simulink model "turbo_controller"  (R2025a)
settings: Solver=FixedStepAuto  StartTime=0.0  StopTime=inf  FixedStep=0.001  RelTol=1e-3
PostLoadFcn:
  | % 自动定位同目录CubeMX文件；不需要外部初始化脚本。
  | codertarget.data.setParameterValue('turbo_controller','STM32CubeMX.ProjectFile',fullfile(fileparts(get_param('turbo_controller','FileName')),'turbo_f407.ioc'));
InitFcn:
  | % 中文说明：按原控制器字段与类型创建三组接口总线；控制参数已内嵌。
  | tc_names=["EValve_Cycle" "EValve_Open" "Eblast_Cycle" "Eblast_Open" "Motor_Cycle" "Motor_Open" "EValve_Enable" "Eblast_Enable" "Motor_Enable" "SWO_Firework" "SWO_BleedAir" "EngineState" "Flag_ECUReset_Clear" "Flag_ECUReset_Save" "Flag_Reset_Enable" "Accelerator" "Nc_dem" "Nc"]; tc_types=["uint16" "uint16" "uint16" "uint16" "uint16" "uint16" "uint8" "uint8" "uint8" "uint8" "uint8" "uint8" "uint8" "uint8" "uint8" "single" "single" "single"];
  | for tc_k=1:numel(tc_names)
  |  tc_e(tc_k)=Simulink.BusElement; tc_e(tc_k).Name=char(tc_names(tc_k)); tc_e(tc_k).DataType=char(tc_types(tc_k));
  | end
  | EngineControl_Out=Simulink.Bus; EngineControl_Out.DataScope='Exported'; EngineControl_Out.Elements=tc_e;
  | clear tc_e tc_names tc_types tc_k
  | tc_names=["savedata1" "savedata2" "savedata3" "savedata4" "savedata5" "savedata6" "savedata7" "savedata8" "savedata9" "savedata10" "savedata11" "savedata12" "savedata13" "savedata14" "savedata15" "savedata16" "savedata17" "savedata18" "savedata19" "savedata20" "savedata21" "savedata22" "savedata23" "savedata24" "savedata25"]; tc_types=["single" "single" "single" "single" "single" "single" "single" "single" "single" "single" "single" "single" "single" "single" "single" "single" "single" "single" "single" "single" "single" "single" "single" "single" "single"];
  | for tc_k=1:numel(tc_names)
  |  tc_e(tc_k)=Simulink.BusElement; tc_e(tc_k).Name=char(tc_names(tc_k)); tc_e(tc_k).DataType=char(tc_types(tc_k));
  | end
  | SaveData_Out=Simulink.Bus; SaveData_Out.DataScope='Exported'; SaveData_Out.Elements=tc_e;
  | clear tc_e tc_names tc_types tc_k
  | tc_names=["senddata1" "senddata2" "senddata3" "senddata4" "senddata5" "senddata6" "senddata7" "senddata8" "senddata9" "senddata10" "senddata11" "senddata12" "senddata13" "senddata14" "senddata15" "senddata16" "senddata17" "senddata18" "senddata19" "senddata20" "senddata21" "senddata22" "senddata23" "senddata24" "senddata25" "senddata26" "senddata27" "senddata28" "senddata29"]; tc_types=["uint8" "uint8" "uint8" "uint8" "uint8" "uint8" "uint8" "uint8" "uint8" "uint8" "uint8" "uint8" "uint8" "uint8" "uint8" "uint8" "uint8" "uint8" "uint8" "uint8" "uint8" "uint8" "uint8" "uint8" "uint8" "uint8" "uint8" "uint8" "uint8"];
  | for tc_k=1:numel(tc_names)
  |  tc_e(tc_k)=Simulink.BusElement; tc_e(tc_k).Name=char(tc_names(tc_k)); tc_e(tc_k).DataType=char(tc_types(tc_k));
  | end
  | SendData_Out=Simulink.Bus; SendData_Out.DataScope='Exported'; SendData_Out.Elements=tc_e;
  | clear tc_e tc_names tc_types tc_k
  | 
  | % 以下为接口中文说明；只设置描述，不改变数值或数据类型。
  | EngineControl_Out.Description='执行控制输出（阀、电机、点火、状态及复位请求）';
  | tc_cn=["EValve_Cycle（主油阀周期计数（每计数2毫秒））" "EValve_Open（主油阀开通计数（每计数2毫秒））" "Eblast_Cycle（副油阀周期计数（每计数2毫秒））" "Eblast_Open（副油阀开通计数（每计数2毫秒））" "Motor_Cycle（起动电机周期计数）" "Motor_Open（起动电机开通计数）" "EValve_Enable（主油阀驱动使能）" "Eblast_Enable（副油阀驱动使能）" "Motor_Enable（起动电机使能）" "SWO_Firework（点火器使能（1开））" "SWO_BleedAir（引气阀使能（1开））" "EngineState（发动机状态）" "Flag_ECUReset_Clear（清除复位恢复状态请求）" "Flag_ECUReset_Save（保存复位恢复数据请求）" "Flag_Reset_Enable（处理器软件复位请求）" "Accelerator（油门／油泵给定控制量）" "Nc_dem（控制目标转速）" "Nc（发动机反馈转速（转每分））"];
  | tc_elements=EngineControl_Out.Elements;
  | for tc_k=1:numel(tc_cn)
  |  tc_elements(tc_k).Description=char(tc_cn(tc_k));
  | end
  | EngineControl_Out.Elements=tc_elements;
  | clear tc_cn tc_elements tc_k
  | SaveData_Out.Description='25项运行记录；字段含义按当前模型数据来源解释';
  | tc_cn=["savedata1（指令回显记录）" "savedata2（入口总温记录（℃））" "savedata3（电源电压记录）" "savedata4（排气温度记录（℃））" "savedata5（标定燃油压力记录）" "savedata6（副油阀占空比记录（％））" "savedata7（主油阀占空比记录（％））" "savedata8（温度修正转速记录）" "savedata9（开关输出及反馈位域）" "savedata10（物理转速记录）" "savedata11（油泵目标给定原始值）" "savedata12（起动电机占空比记录（％））" "savedata13（发动机状态码记录）" "savedata14（故障告警位域记录）" "savedata15（模型记录帧序号）" "savedata16（处理器温度记录（℃））" "savedata17（装订转速记录（沿用旧电源字段名））" "savedata18（导航高度记录）" "savedata19（飞行空速记录）" "savedata20（主阀旧记录位（恒零保留））" "savedata21（第21项保留记录（恒零））" "savedata22（保留记录项22）" "savedata23（保留记录项23）" "savedata24（保留记录项24）" "savedata25（保留记录项25）"];
  | tc_elements=SaveData_Out.Elements;
  | for tc_k=1:numel(tc_cn)
  |  tc_elements(tc_k).Description=char(tc_cn(tc_k));
  | end
  | SaveData_Out.Elements=tc_elements;
  | clear tc_cn tc_elements tc_k
  | SendData_Out.Description='29字段回传及外设命令接口；板端上位机帧只取第3至27字段';
  | tc_cn=["senddata1（回传发送允许标志（不直接上线路））" "senddata2（回传载荷长度25字节）" "senddata3（回传指令回显字节）" "senddata4（总温编码字节（℃＋80））" "senddata5（电源电压编码字节）" "senddata6（排温编码高字节）" "senddata7（排温编码低字节）" "senddata8（燃油压力编码高字节）" "senddata9（燃油压力编码低字节）" "senddata10（副油阀占空比字节（％））" "senddata11（主油阀占空比字节（％））" "senddata12（修正转速编码高字节）" "senddata13（修正转速编码低字节）" "senddata14（驱动及反馈状态位域）" "senddata15（物理转速编码高字节）" "senddata16（物理转速编码低字节）" "senddata17（油泵目标给定高字节（串口二使用））" "senddata18（油泵目标给定低字节（串口二使用））" "senddata19（起动电机占空比命令（串口一使用））" "senddata20（发动机状态码字节）" "senddata21（故障告警位域字节）" "senddata22（帧序号占位（板端另行填写））" "senddata23（处理器温度编码（℃＋50））" "senddata24（控制目标转速编码高字节）" "senddata25（控制目标转速编码低字节）" "senddata26（占位字节（板端改填实测泵速高字节））" "senddata27（占位字节（板端改填实测泵速低字节））" "senddata28（装订转速高字节（本板未发送））" "senddata29（装订转速低字节（本板未发送））"];
  | tc_elements=SendData_Out.Elements;
  | for tc_k=1:numel(tc_cn)
  |  tc_elements(tc_k).Description=char(tc_cn(tc_k));
  | end
  | SendData_Out.Elements=tc_elements;
  | clear tc_cn tc_elements tc_k
  | 
  | 
  | % FRAM模块化事务：接口类型和上电初始状态，随模型保存，无外部初始化文件。
  | clear FM_elements
  | FM_elements(1)=Simulink.BusElement;FM_elements(1).Name='phase';FM_elements(1).DataType='uint8';FM_elements(1).Dimensions=[1 1];FM_elements(1).Description='phase（当前事务阶段）';
  | FM_elements(2)=Simulink.BusElement;FM_elements(2).Name='a';FM_elements(2).DataType='uint8';FM_elements(2).Dimensions=[64 1];FM_elements(2).Description='a（启动时缓存的首区64字节）';
  | FM_elements(3)=Simulink.BusElement;FM_elements(3).Name='active';FM_elements(3).DataType='uint16';FM_elements(3).Dimensions=[1 1];FM_elements(3).Description='active（当前有效记录区地址）';
  | FM_elements(4)=Simulink.BusElement;FM_elements(4).Name='generation';FM_elements(4).DataType='uint32';FM_elements(4).Dimensions=[1 1];FM_elements(4).Description='generation（当前有效记录代号）';
  | FM_elements(5)=Simulink.BusElement;FM_elements(5).Name='record';FM_elements(5).DataType='uint8';FM_elements(5).Dimensions=[64 1];FM_elements(5).Description='record（本次冻结的待写记录）';
  | FM_elements(6)=Simulink.BusElement;FM_elements(6).Name='addr';FM_elements(6).DataType='uint16';FM_elements(6).Dimensions=[1 1];FM_elements(6).Description='addr（本次备用写入地址）';
  | FM_elements(7)=Simulink.BusElement;FM_elements(7).Name='lastSave';FM_elements(7).DataType='single';FM_elements(7).Dimensions=[1 1];FM_elements(7).Description='lastSave（上次开始保存的秒数）';
  | FM_elements(8)=Simulink.BusElement;FM_elements(8).Name='lastState';FM_elements(8).DataType='uint8';FM_elements(8).Dimensions=[1 1];FM_elements(8).Description='lastState（上次保存时的发动机状态）';
  | FM_elements(9)=Simulink.BusElement;FM_elements(9).Name='boot';FM_elements(9).DataType='boolean';FM_elements(9).Dimensions=[1 1];FM_elements(9).Description='boot（启动记录是否允许恢复）';
  | FM_elements(10)=Simulink.BusElement;FM_elements(10).Name='consumed';FM_elements(10).DataType='boolean';FM_elements(10).Dimensions=[1 1];FM_elements(10).Description='consumed（本次启动恢复通知是否已发送）';
  | FM_elements(11)=Simulink.BusElement;FM_elements(11).Name='payload';FM_elements(11).DataType='uint8';FM_elements(11).Dimensions=[20 1];FM_elements(11).Description='payload（当前20字节恢复内容）';
  | ... (+35 lines)
model workspace (MAT data in the model file):
  CRC16_Table_Reference = [0 4129 8258 12387 16516 20645 24774 28903 33032 37161 41290 45419 ... (256 elements, 256x1)]
  PE_Kaer = [0.15402 0.15402 0.12264 0.10076 0.09481 0.07601 0.07111 0.0569 0.05198 0.04926 0.05308 0.04325 ... (13 elements, 1x13)]
  PE_Nr = [21.2982 61.4260372 67.7475458 72.7394382 76.845934 80.6988798 83.8449282 86.6491912 88.9382406 89.178606 91.1938214 93.4068058 ... (13 elements, 1x13)]
  PE_Pump_Translate = 33.5999984741
  PE_RotaSpeed_Translate = 860
  PE_Taer = [0.4939154 0.4939154 0.40780982 0.34066978 0.31622756 0.30405716 0.34300244 0.26785022 0.37393554 0.23914836 0.44563948 0.31044662 ... (13 elements, 1x13)]
  PF_ACCFULLRANGE = 3360
  PF_Flag_ECUReset = 0
  PF_Flag_rx_suc = 1
  PF_Gear_Info = [40000; 45000; 50000; 55000; 57000; 59000; 60000; 61000; 61000; 61000; 61000; 61000]
  PF_K_TiaoJie = 1
  PF_Kpu = 10
  PF_MySet_Rxdata = [0 0 0 0 0 0 0 0 0 0 0 0 ... (50 elements, 50x1)]
  PF_MyUsart1_Rxdata = [0 0 0 0 0 0 0 0 0 0 0 0 ... (50 elements, 50x1)]
  PF_MyUsart2_Rxdata = [0 0 0 0 0 0 0 0 0 0 0 0 ... (50 elements, 50x1)]
  PF_Reset_Information = [0 0 0 0 0 0 0 0 0 0 0 0 ... (20 elements, 20x1)]
  PF_Sensor_X1_T4 = [0 4095]
  PF_Sensor_X2_T4 = [0 1.66666698456]
  PF_Sensor_X3_T4 = [0 504 999 1497 2010 2529 3051 3568 4076 4571 4959]
  PF_Sensor_X_P2 = [0.5 3]
  PF_Sensor_X_Poil = [0.5 3]
  PF_Sensor_X_T1t = [-50 300]
  PF_Sensor_X_Vpower = [0 3]
  PF_Sensor_X_Vpump = [0 3]
  PF_Sensor_Y1_T4 = [0 3]
  PF_Sensor_Y2_T4 = [0 5000]
  PF_Sensor_Y3_T4 = [0 100 200 300 400 500 600 700 800 900 980]
  PF_Sensor_Y_P2 = [0 1000]
  PF_Sensor_Y_Poil = [0 1000]
  PF_Sensor_Y_T1t = [-50 300]
  PF_Sensor_Y_Vpower = [0 33]
  PF_Sensor_Y_Vpump = [0 33]
  PG_CtrlMode_CloseLoop : mpt.Parameter (value not decoded)
  PG_CtrlMode_ManualAcc : mpt.Parameter (value not decoded)
  PG_CtrlMode_Origin : mpt.Parameter (value not decoded)
  PG_CtrlMode_Start : mpt.Parameter (value not decoded)
  PG_CtrlMode_Stop : mpt.Parameter (value not decoded)
  PG_ES_Clp : mpt.Parameter (value not decoded)
  PG_ES_EngStart : mpt.Parameter (value not decoded)
  PG_ES_Manual : mpt.Parameter (value not decoded)
  PG_ES_Origin : mpt.Parameter (value not decoded)
  PG_ES_Stop : mpt.Parameter (value not decoded)
  PG_Instr_BleedAirSet : mpt.Parameter (value not decoded)
  PG_Instr_CloseLoop : mpt.Parameter (value not decoded)
  PG_Instr_ECUReSet : mpt.Parameter (value not decoded)
  PG_Instr_EValveSet : mpt.Parameter (value not decoded)
  PG_Instr_EblastSet : mpt.Parameter (value not decoded)
  PG_Instr_Erase : mpt.Parameter (value not decoded)
  PG_Instr_FireWorkSet : mpt.Parameter (value not decoded)
  PG_Instr_ManualPlus : mpt.Parameter (value not decoded)
  PG_Instr_ManualrReduce : mpt.Parameter (value not decoded)
  PG_Instr_MotorSet : mpt.Parameter (value not decoded)
  PG_Instr_OilSet : mpt.Parameter (value not decoded)
  PG_Instr_SelfCheck : mpt.Parameter (value not decoded)
  PG_Instr_Start : mpt.Parameter (value not decoded)
  PG_Instr_Stop : mpt.Parameter (value not decoded)
  PG_Instr_StopZero : Simulink.Parameter (value not decoded)
  PG_Location_Air : Simulink.Parameter (value not decoded)
  PG_Location_Gnd : Simulink.Parameter (value not decoded)
  PG_ServoCtrlMode_CloseLoop : Simulink.Parameter (value not decoded)
  PG_ServoCtrlMode_CloseLoopMax : Simulink.Parameter (value not decoded)
  PG_ServoCtrlMode_CloseLoopMin : Simulink.Parameter (value not decoded)
  PG_ServoCtrlMode_ManualAcc : Simulink.Parameter (value not decoded)
  PG_ServoCtrlMode_ManualAccMax : Simulink.Parameter (value not decoded)
  PG_ServoCtrlMode_ManualAccMin : Simulink.Parameter (value not decoded)
  PG_SpeedDot_Permit : Simulink.Parameter (value not decoded)
  PL_EngineModel_Actuator = [0 10 100]
  PL_EngineModel_EngineStar_Press_P2 = [1013 1098.4 1099.144828 1099.931034 1103.613793 1162.662069 1143.793103 1131.006897 1123.186207 1117.6 1114 1111.806897 ... (127 elements, 1x127)]
  PL_EngineModel_EngineStar_RotaSpeed = [200 2000 9584 9660 10220 10240 10260 10288 10308 10368 10380 10408 ... (127 elements, 1x127)]
  PL_EngineModel_EngineStar_Temp_Exhaust = [128 129 129.1 130 131 131.1 132 133 134 134.1 135 135.1 ... (127 elements, 1x127)]
  PL_EngineModel_EngineStar_Time = [0.05 0.1 0.15 0.2 0.25 0.3 0.35 0.4 0.45 0.5 0.55 0.6 ... (127 elements, 1x127)]
  PL_EngineModel_IdleAbove_Nr = [0 21.2982 61.4260372 67.7475458 72.7394382 76.845934 80.6988798 83.8449282 86.6491912 88.9382406 89.178606 91.1938214 ... (14 elements, 1x14)]
  PL_EngineModel_IdleAbove_P2r = [0.986923266716 1.57907722675 1.81593881076 1.99358499877 2.23044658278 2.43770046879 2.65482358747 2.84233900814 3.03972366149 3.18776215149 3.25684678016 3.3950160375 ... (14 elements, 1x14)]
  PL_EngineModel_IdleAbove_Tempr = [0.0536001429337 1.07200285867 1.63301768805 1.63659103091 1.66875111667 1.72592460247 1.77595140254 1.86171163123 1.95461854565 2.03323208862 2.03323208862 2.13685903162 ... (14 elements, 1x14)]
  PL_EngineModel_IdleAbove_Ter = [0.42434128 0.42434128 0.42434128 0.30669408 0.23570008 0.22150128 0.1997974 0.23803274 0.16115638 0.24279948 0.13600422 0.31308354 ... (14 elements, 1x14)]
  PL_EngineModel_IdleAbove_Wfr = [0 10.142 23.8337 27.8905 31.9473 36.0041 40.0609 44.1177 48.1745 52.2313 52.7384 56.7952 ... (14 elements, 1x14)]
  PL_EngineModel_Press_P2 = [400 400 400 400 400 400 400 400 400 400]
  PL_EngineModel_Rotaspeed = [0 20000 96400]
  PL_EngineModel_Temp_Exhaust = [500 500 500 500 500 500 500 500 500 500]
  PL_Kaer = [0.1 0.1 0.1 0.1 0.1 0.1]
  PL_Nr = [50 60 70 80 90 100]
  PL_Taer = [0.1 0.1 0.1 0.1 0.1 0.1]
  Sig : Simulink.Signal (value not decoded)
  Ts_ms : Simulink.Parameter (value not decoded)
  false : Simulink.Parameter (value not decoded)
  true : Simulink.Parameter (value not decoded)
symbols that are objects in the model workspace (value not decoded): PG_CtrlMode_CloseLoop, PG_CtrlMode_ManualAcc, PG_CtrlMode_Origin, PG_CtrlMode_Start, PG_CtrlMode_Stop, PG_ES_Clp, PG_ES_EngStart, PG_ES_Manual, PG_ES_Origin, PG_ES_Stop, PG_Instr_BleedAirSet, PG_Instr_CloseLoop, PG_Instr_EblastSet, PG_Instr_ECUReSet, PG_Instr_Erase, PG_Instr_EValveSet, PG_Instr_FireWorkSet, PG_Instr_ManualPlus, PG_Instr_ManualrReduce, PG_Instr_MotorSet, PG_Instr_OilSet, PG_Instr_SelfCheck, PG_Instr_Start, PG_Instr_Stop, PG_Instr_StopZero, PG_ServoCtrlMode_CloseLoop, PG_ServoCtrlMode_CloseLoopMax, PG_ServoCtrlMode_CloseLoopMin, PG_ServoCtrlMode_ManualAcc, PG_ServoCtrlMode_ManualAccMax, PG_ServoCtrlMode_ManualAccMin, Ts_ms
libraries: simulink x97, stm32blockslib x10, stm32f4xxblockslib x8
(part 21 of 26)

== system turbo_controller/BoardInput_输入换算与协议解析/In01_Host（上位机命令解析）/Receive（逐字节组帧与保持有效结果）_108/Step03_检查完整性与双校验/Verify（完整帧校验）_93 ==
  note: 上位机候选帧怎样通过最后检查
      |
      | Collect已经收齐14字节后，本模块才开始检查。Complete转成0或1次的执行许可：不完整时不重新计
      | 算，以免读到半帧；完整时取协议规定的数据段，同时计算累加与异或校验。
      |
      | Checksum中两种规则分别为：
      | 累加校验 = 所有待校验字节之和对256取余；
      | 异或校验 = 所有待校验字节逐个按位异或。
      | 计算出的两项分别与候选帧尾部校验项比较，两项都相同才输出通过。
      |
      | 校验失败时，外层Receive保留旧命令，等待下一帧。外层还把“校验通过”和“本次刚收齐”组合，
      | 避免把上次通过的保持值误当成本次新帧也通过。
      |
      | 这里不解释FC、F0等命令含义；命令解码要等数据可靠之后交给CMMRead/Instr_Analyse。
      |
      | 本实例对第1～12字节计算累加和及异或值，分别与第13、第14字节比较。
  Complete（完整帧执行一次）_67 : Inport  OutDataTypeStr=uint32
  Frame（完整候选帧）_69 : Inport  Port=2  OutDataTypeStr=uint8
  Checksum（累加与异或校验）_85 : Subsystem  Description=|
      | 一段字节怎样得到累加和异或两种校验
      | 
      | 输入是一整段需要校验的字节。每帧开始，两路累积值都从0开始；For Iterator按顺序取出每个字节，同时更新两路结果。
      | 
      | 累加这一路只保留低8位：
      | 新累加值 = mod(旧累加值 + 当前字节,256)。
      | 例如三个字节为200、100、1，总和301，最后校验字节为45，不让普通uint8溢出替代明确的取余规则。
      | 
      | 异或这一路逐位计算：
      | 新异或值 = bitxor(旧异或值,当前字节)。
      | 相同比特异或得到0，不同比特得到1。它与“所有数相加”是两种不同检查。
      | 
      | 接收侧拿这两个结果和帧尾比较，发送侧把结果追加到帧尾。父级负责规定哪些字节参加计算；本模块不验证帧头，也不能替换电机/油泵协议使用的CRC16。
  FirstCheck（第一个校验字节一致）_87 : RelationalOperator  Operator===  OutDataTypeStr=boolean  RndMeth=Simplest  InputSameDT=off
  Payload（参与累加异或的字节）_70 : Selector  InputPortWidth=14  IndexOptions=Index vector (dialog)  Indices=1:12  OutputSizes=1
  SecondCheck（第二个校验字节一致）_89 : RelationalOperator  Operator===  OutDataTypeStr=boolean  RndMeth=Simplest  InputSameDT=off
  Select（取指定元素）_86 : Selector  InputPortWidth=14  IndexOptions=Index vector (dialog)  Indices=13  OutputSizes=1
  Select（取指定元素）_88 : Selector  InputPortWidth=14  IndexOptions=Index vector (dialog)  Indices=14  OutputSizes=1
  Valid（两个校验字节均正确）_90 : Logic  IconShape=distinctive  AllPortsSameDT=off  OutDataTypeStr=boolean
  WhenComplete（完整帧才执行一次）_68 : ForIterator  IterationSource=external  ShowIterationPort=off
  Valid（校验是否通过）_91 : Outport
  wires:
  Complete（完整帧执行一次）_67/1 -> WhenComplete（完整帧才执行一次）_68/1  "Complete（完整帧执行一次）"
  Frame（完整候选帧）_69/1 -> Select（取指定元素）_86/1, Payload（参与累加异或的字节）_70/1, Select（取指定元素）_88/1  "Frame（完整候选帧）"
  Payload（参与累加异或的字节）_70/1 -> Checksum（累加与异或校验）_85/1(Bytes（待校验字节）_71)  "Payload（参与累加异或的字节）"
  Checksum（累加与异或校验）_85/1(Sum8（八位累加结果）_83) -> FirstCheck（第一个校验字节一致）_87/1  "Checksum（累加与异或校验）"
  Select（取指定元素）_86/1 -> FirstCheck（第一个校验字节一致）_87/2  "Select（取指定元素）"
  Checksum（累加与异或校验）_85/2(Xor8（八位异或结果）_84) -> SecondCheck（第二个校验字节一致）_89/1  "Checksum（累加与异或校验）"
  Select（取指定元素）_88/1 -> SecondCheck（第二个校验字节一致）_89/2  "Select（取指定元素）"
  FirstCheck（第一个校验字节一致）_87/1 -> Valid（两个校验字节均正确）_90/1  "FirstCheck（第一个校验字节一致）"
  SecondCheck（第二个校验字节一致）_89/1 -> Valid（两个校验字节均正确）_90/2  "SecondCheck（第二个校验字节一致）"
  Valid（两个校验字节均正确）_90/1 -> Valid（校验是否通过）_91/1  "Valid（两个校验字节均正确）"

== system turbo_controller/BoardInput_输入换算与协议解析/In02_Motor（电机反馈解析）/Receive（逐字节组帧与保持有效结果）_235/Step02_拼帧并保存半帧/Collect（帧头识别与缓存推进）_167 ==
  note: 逐字节组帧：本页只做“找帧头、存字节、推进位置”
      |
      | 固定帧长为9字节，帧头是十六进制AA、55。输入为上一份候选缓存、已收字节数Position、本次Byte
      | 和本字节有效Active。输出为更新缓存、下一次使用的Position和本次收齐事件Complete。
      |
      | Position不是本批接收数组的序号：0表示还在找AA，1表示已见AA、正在等55，2～8表示头部已确认、
      | 继续收后面的内容。跨调用的记忆由外层Step02保存，本页根据输入计算一次更新。
      |
      | 按五步看：
      | 1 判断当前是否在等AA或55，以及字节是否匹配。
      | 2 决定这个字节应不应该进入候选缓存。
      | 3 算出本次写入位置Position+1，判断是否达到9。
      | 4 允许写入才更新对应一项，否则保留原缓存。
      | 5 按找头、重同步、收齐和无效字节规则，决定下一位置及Complete。
      |
      | 例：AA→AA→55时，第二个AA保留继续等55的机会，不当作第二帧头写入；头确认后，后续数据即使也
      | 是AA或55，仍按普通数据收下。无效字节不推进位置，也不发收齐事件。
      |
      | Complete仅表示候选帧刚拼满，不表示校验通过；外面的校验步骤还会检查内容。这里没有重写协议或
      | 增加等待时间，五步在同一次字节处理内完成。
  Buffer（上次收帧缓存）_128 : Inport  OutDataTypeStr=uint8
  Position（已收字节数）_129 : Inport  Port=2  OutDataTypeStr=uint16
  Byte（当前字节）_130 : Inport  Port=3  OutDataTypeStr=uint8
  Active（当前字节有效）_131 : Inport  Port=4  OutDataTypeStr=boolean
  Step01_判断收帧阶段与AA55 : Subsystem  Description=|
      | 第一步：看现在收到哪里，并识别AA、55
      | 
      | 只看Position和Byte，不修改缓存，不保存历史。输出三个判断：是否正在找第一个AA、当前字节是否AA、是否发生第二帧头不匹配。
      | 
      | Position=0：还没确认帧头，正在找AA。
      | Position=1：已经见到AA，期望下一个是55。
      | Position≥2：头部已确认，后续字节属于帧内数据。
      | 
      | AA是十六进制，十进制为170；55是十六进制，十进制为85。判断式：
      | 等待AA=(Position==0)；
      | 字节是AA=(Byte==170)；
      | 第二帧头错=(Position==1) AND (Byte!=85)。
      | 
      | 例：Position=1、Byte=AA时，字节是AA和第二帧头错都为真。这并不冲突：它表示没等到55，但可以把这个AA视作重新找头的机会。是否写入、位置如何调整由后面两步分别处理。
      | 
      | 本步骤不检查Active；本字节无效时，后面的写入和位置保持分支会阻止它改变状态。
  Step02_判断本字节能否写入 : Subsystem  Description=|
      | 第二步：决定本字节是否允许写进帧缓存
      | 
      | 收帧必须先找到头，所以不是每个字节都写。将第一步的三个判断与Active组合：
      | 
      | 允许写入=Active AND [
      |   (正在等AA AND 字节是AA)
      |   OR (不在等AA AND 第二帧头没有错)
      | ]。
      | 
      | 分别理解：
      | 还在找AA时，只写AA，其他噪声不进入缓存；
      | 已经见到AA、等待55时，只写正确的55；
      | 头部已经确认后，按顺序接收普通数据，不因数据恰好是AA/55就重新找头；
      | Active为假时，上述条件再合适也不写。
      | 
      | 例：已见AA后又来AA，本步骤不把第二个AA写进第2项；后面的重同步位置逻辑仍保留“已见AA”的状态，继续等55。
      | 
      | 输出只是一项布尔写许可，送第四步。它不产生新缓存，也不判断整帧校验。
  Step03_计算写入位置与是否满帧 : Subsystem  Description=|
      | 第三步：算本次写到第几项，并判断是否到帧尾
      | 
      | Position表示本次之前已接收多少项。本次候选写入位置=Position+1；帧长度固定为9，达到帧尾=(候选写入位置==9)。
      | 
      | 例如Position=0时，候选位置是1，AA应写到第1项；Position=1时，55应写到第2项；Position=8时，本次候选位置是9，这是最后一项。
      | 
      | 注意这里算的是“候选位置”：即使Active为假，仍可计算Position+1，但第四、第五步会保持缓存和位置。不能仅因候选位置等于9就认定收到新帧。
      | 
      | 候选位置送第四步写缓存；它及“达到帧尾”标志也送第五步，决定继续推进还是收齐后回0。本处不保存Position，也不清空缓存。
  Step04_写入字节或保持原缓存 : Subsystem  Description=|
      | 第四步：只更新应写的一项，其他内容保留
      | 
      | 输入包括旧缓存、本次Byte、候选写入位置和写许可。先将索引取min(候选位置,9)，防止索引超过9项缓存上界，再用Assignment生成“把这一项换成Byte”的候选数组。
      | 
      | 最终选择：写许可为真输出更新数组；写许可为假直接输出旧缓存。即使内部算出了候选更新，只要没有许可，它也不会成为输出。
      | 
      | 例：旧位置为5，本次允许接收，就把第6项换成本字节，其他8项保持；若本字节无效或第二帧头错，整份缓存保持。缓存里旧的尾部数据并不会每次清零，所以必须配合Complete和后续校验使用，不能只看数组里有值就当作新帧。
      | 
      | 本步骤不保存跨调用记忆。输出回外层的缓存记忆，供下一个字节/下一批数据继续使用。位置更新与收齐事件在第五步处理。
  Step05_更新收帧位置并报告收齐 : Subsystem  Description=|
      | 第五步：确定下一次收帧位置，并报告刚收齐
      | 
      | 先按收帧阶段选择下一Position：
      | 正在找AA：本字节是AA则到1，否则到0；
      | 正在等55但本字节不匹配：若又是AA则保持1，其他值回0；
      | 正常收数据：未到帧尾就采用Position+1，达到9项后回0，准备找下一帧头。
      | 最后再检查Active：为假时直接保留旧Position，上面的候选变化都不采用。
      | 
      | 收齐事件=Active AND 不在等待第一个AA AND 第二帧头没错 AND 达到9项。
      | 因此它只在有效字节刚补上最后一项时为真，不是缓存里有9项就一直为真。位置回0时，完整缓存仍保留供外层校验。
      | 
      | 例：Position=8，有效字节到来，输出Position=0且Complete=true；同样的位置但Active=false，则输出仍为8且Complete=false。AA、AA、55的序列依次得到位置1、1、2。
      | 
      | 本页不验证CRC或累加/异或校验，也不等待下一个20 ms节拍；Complete交外层决定是否接受这条候选帧。
  Buffer（更新后的帧缓存）_164 : Outport
  Position（下次接收位置）_165 : Outport  Port=2
  Complete（本字节组成完整帧）_166 : Outport  Port=3
  wires:
  Step05_更新收帧位置并报告收齐/1(输出1_下一次已收字节数) -> Position（下次接收位置）_165/1
  Byte（当前字节）_130/1 -> Step04_写入字节或保持原缓存/4(输入4_本项字节), Step01_判断收帧阶段与AA55/1(输入1_本项字节)  "本项字节"
  Active（当前字节有效）_131/1 -> Step02_判断本字节能否写入/4(输入4_本项字节有效), Step05_更新收帧位置并报告收齐/2(输入2_本项字节有效)  "本项字节有效"
  Step02_判断本字节能否写入/1(输出1_本字节允许写缓存) -> Step04_写入字节或保持原缓存/1(输入1_本字节允许写缓存)  "本字节允许写缓存"
  Position（已收字节数）_129/1 -> Step05_更新收帧位置并报告收齐/5(输入5_本次之前已收字节数), Step03_计算写入位置与是否满帧/1(输入1_本次之前已收字节数), Step01_判断收帧阶段与AA55/2(输入2_本次之前已收字节数)  "本次之前已收字节数"
  Step03_计算写入位置与是否满帧/1(输出1_候选位置达到帧长) -> Step05_更新收帧位置并报告收齐/3(输入3_候选位置达到帧长)  "候选位置达到帧长"
  Step01_判断收帧阶段与AA55/2(输出2_正在寻找第一个AA) -> Step05_更新收帧位置并报告收齐/6(输入6_正在寻找第一个AA), Step02_判断本字节能否写入/1(输入1_正在寻找第一个AA)  "正在寻找第一个AA"
  Step01_判断收帧阶段与AA55/1(输出1_当前字节等于AA) -> Step05_更新收帧位置并报告收齐/1(输入1_当前字节等于AA), Step02_判断本字节能否写入/2(输入2_当前字节等于AA)  "当前字节等于AA"
  Step01_判断收帧阶段与AA55/3(输出3_第二帧头不匹配) -> Step05_更新收帧位置并报告收齐/7(输入7_第二帧头不匹配), Step02_判断本字节能否写入/3(输入3_第二帧头不匹配)  "第二帧头不匹配"
  Step03_计算写入位置与是否满帧/2(输出2_候选写入位置) -> Step04_写入字节或保持原缓存/3(输入3_候选写入位置), Step05_更新收帧位置并报告收齐/4(输入4_候选写入位置)  "候选写入位置"
  Buffer（上次收帧缓存）_128/1 -> Step04_写入字节或保持原缓存/2(输入2_上一份候选缓存)  "上一份候选缓存"
  Step05_更新收帧位置并报告收齐/2(输出2_本字节刚收齐) -> Complete（本字节组成完整帧）_166/1
  Step04_写入字节或保持原缓存/1(输出1_更新后的候选缓存) -> Buffer（更新后的帧缓存）_164/1

== system turbo_controller/BoardInput_输入换算与协议解析/In02_Motor（电机反馈解析）/Receive（逐字节组帧与保持有效结果）_235/Step03_收齐且校验通过才接受/Verify（完整帧校验）_218 ==
  note: 电机9字节反馈怎样核对CRC
      |
      | Collect送来的是候选完整帧，本模块只在Complete有效时执行校验。内部取协议指定的待校验字节段
      | ，送CRC16逐字节计算，并取出帧尾携带的两个CRC字节。
      |
      | 16位计算结果分为高低两部分：高字节=floor(CRC/256)，低字节=bitand(CRC,255)。分别与帧中对应
      | 位置比较，两项都一致才给出有效结果。
      |
      | 比如计算CRC为十六进制1234，协议中的CRC高字节必须是12、低字节必须是34；顺序反过来也不能通过
      | 。CRC覆盖范围由本页Selector的固定索引决定，不应把帧头或尾部CRC自身随意加入。
      |
      | 输出交给Receive，与“这一轮确实刚收齐一帧”共同决定是否更新反馈。不完整或校验错误时，外层
      | 保留最近有效结果。
      |
      | 本实例CRC覆盖第6～7字节，接收的CRC高、低字节在第8、9字节。
  Complete（完整帧执行一次）_168 : Inport  OutDataTypeStr=uint32
  Frame（完整候选帧）_170 : Inport  Port=2  OutDataTypeStr=uint8
  CRC16（循环冗余校验）_202 : Subsystem  Description=|
      | 整段字节如何逐个累积CRC16
      | 
      | 这里的输入Bytes是接收帧中由父级Selector选出的数据段。CRC的作用是把整段字节压缩成一个16位检查值，便于接收方发现传输内容变化。
      | 
      | 每帧从初始CRC=uint16(0)开始。循环一次取一个字节，把该字节乘256移到高8位，与旧CRC异或，得到Merged，再交给TableStep执行查表移位。TableStep的输出成为处理下一个字节的旧CRC。
      | 
      | 公式第一步是Merged=bitxor(旧CRC,当前字节×256)。整个循环结束后输出最后一次CRC，父级拆成高、低字节用于比较或发送。For Iterator中的CRC记忆是帧内累积状态，不能理解成跨帧无限累加。
      | 
      | 这里用的是CRC16_Table_Reference指定的算法表，不能随意换另一种CRC表或初始值。相同字节、顺序、表和初值必须得到相同结果，双方才能校验通过。
  Cast（数据类型转换）_203 : DataTypeConversion  OutDataTypeStr=double  RndMeth=Round
  Constant（常量）_204 : Constant  Value=256  OutDataTypeStr=double
  Constant（常量）_208 : Constant  Value=255  OutDataTypeStr=uint16
  Divide（相除）_205 : Product  Inputs=*/  SaturateOnIntegerOverflow=on  OutDataTypeStr=Inherit: Same as first input
  FirstCheck（第一个校验字节一致）_212 : RelationalOperator  Operator===  OutDataTypeStr=boolean  RndMeth=Simplest  InputSameDT=off
  HighByte（高八位）_207 : DataTypeConversion  OutDataTypeStr=uint8  RndMeth=Floor
  LowByte（低八位）_210 : DataTypeConversion  OutDataTypeStr=uint8  RndMeth=Floor
  LowMask（取低八位）_209 : simulink/Logic and Bit Operations/Bitwise Operator  logicop=AND  UseBitMask=off  NumInputPorts=2  BitMask=bin2dec('11011001')  BitMaskRealWorld=Stored Integer
      settings: LibrarySourceBlock=|
      | hdlsllib/Logic and Bit
      | Operations/Bitwise
      | Operator
  Payload（参与循环冗余校验的字节）_171 : Selector  InputPortWidth=9  IndexOptions=Index vector (dialog)  Indices=6:7  OutputSizes=1
  Round（取整）_206 : Rounding
  SecondCheck（第二个校验字节一致）_214 : RelationalOperator  Operator===  OutDataTypeStr=boolean  RndMeth=Simplest  InputSameDT=off
  Select（取指定元素）_211 : Selector  InputPortWidth=9  IndexOptions=Index vector (dialog)  Indices=8  OutputSizes=1
  Select（取指定元素）_213 : Selector  InputPortWidth=9  IndexOptions=Index vector (dialog)  Indices=9  OutputSizes=1
  Valid（两个校验字节均正确）_215 : Logic  IconShape=distinctive  AllPortsSameDT=off  OutDataTypeStr=boolean
  WhenComplete（完整帧才执行一次）_169 : ForIterator  IterationSource=external  ShowIterationPort=off
  Valid（校验是否通过）_216 : Outport
  wires:
  Constant（常量）_204/1 -> Divide（相除）_205/2  "Constant（常量）"
  Constant（常量）_208/1 -> LowMask（取低八位）_209/2  "Constant（常量）"
  Frame（完整候选帧）_170/1 -> Payload（参与循环冗余校验的字节）_171/1, Select（取指定元素）_213/1, Select（取指定元素）_211/1  "Frame（完整候选帧）"
  Cast（数据类型转换）_203/1 -> Divide（相除）_205/1  "Cast（数据类型转换）"
  CRC16（循环冗余校验）_202/1(CRC16（本帧校验结果）_201) -> Cast（数据类型转换）_203/1, LowMask（取低八位）_209/1  "CRC16（循环冗余校验）"
  Complete（完整帧执行一次）_168/1 -> WhenComplete（完整帧才执行一次）_169/1  "Complete（完整帧执行一次）"
  Round（取整）_206/1 -> HighByte（高八位）_207/1  "Round（取整）"
  Payload（参与循环冗余校验的字节）_171/1 -> CRC16（循环冗余校验）_202/1(Bytes（待校验字节）_172)  "Payload（参与循环冗余校验的字节）"
  Select（取指定元素）_213/1 -> SecondCheck（第二个校验字节一致）_214/2  "Select（取指定元素）"
  LowMask（取低八位）_209/1 -> LowByte（低八位）_210/1  "LowMask（取低八位）"
  Divide（相除）_205/1 -> Round（取整）_206/1  "Divide（相除）"
  LowByte（低八位）_210/1 -> SecondCheck（第二个校验字节一致）_214/1  "LowByte（低八位）"
  SecondCheck（第二个校验字节一致）_214/1 -> Valid（两个校验字节均正确）_215/2  "SecondCheck（第二个校验字节一致）"
  HighByte（高八位）_207/1 -> FirstCheck（第一个校验字节一致）_212/1  "HighByte（高八位）"
  Select（取指定元素）_211/1 -> FirstCheck（第一个校验字节一致）_212/2  "Select（取指定元素）"
  FirstCheck（第一个校验字节一致）_212/1 -> Valid（两个校验字节均正确）_215/1  "FirstCheck（第一个校验字节一致）"
  Valid（两个校验字节均正确）_215/1 -> Valid（校验是否通过）_216/1  "Valid（两个校验字节均正确）"

== system turbo_controller/BoardInput_输入换算与协议解析/In03_Pump（油泵回包预留校验）/Receive（逐字节组帧与保持有效结果）_353/Step02_拼帧并保存半帧/Collect（帧头识别与缓存推进）_293 ==
  note: 逐字节组帧：本页只做“找帧头、存字节、推进位置”
      |
      | 固定帧长为22字节，帧头是十六进制AA、55。输入为上一份候选缓存、已收字节数Position、本次Byte
      | 和本字节有效Active。输出为更新缓存、下一次使用的Position和本次收齐事件Complete。
      |
      | Position不是本批接收数组的序号：0表示还在找AA，1表示已见AA、正在等55，2～21表示头部已确认
      | 、继续收后面的内容。跨调用的记忆由外层Step02保存，本页根据输入计算一次更新。
      |
      | 按五步看：
      | 1 判断当前是否在等AA或55，以及字节是否匹配。
      | 2 决定这个字节应不应该进入候选缓存。
      | 3 算出本次写入位置Position+1，判断是否达到22。
      | 4 允许写入才更新对应一项，否则保留原缓存。
      | 5 按找头、重同步、收齐和无效字节规则，决定下一位置及Complete。
      |
      | 例：AA→AA→55时，第二个AA保留继续等55的机会，不当作第二帧头写入；头确认后，后续数据即使也
      | 是AA或55，仍按普通数据收下。无效字节不推进位置，也不发收齐事件。
      |
      | Complete仅表示候选帧刚拼满，不表示校验通过；外面的校验步骤还会检查内容。这里没有重写协议或
      | 增加等待时间，五步在同一次字节处理内完成。
  Buffer（上次收帧缓存）_254 : Inport  OutDataTypeStr=uint8
  Position（已收字节数）_255 : Inport  Port=2  OutDataTypeStr=uint16
  Byte（当前字节）_256 : Inport  Port=3  OutDataTypeStr=uint8
  Active（当前字节有效）_257 : Inport  Port=4  OutDataTypeStr=boolean
  Step01_判断收帧阶段与AA55 : Subsystem  Description=|
      | 第一步：看现在收到哪里，并识别AA、55
      | 
      | 只看Position和Byte，不修改缓存，不保存历史。输出三个判断：是否正在找第一个AA、当前字节是否AA、是否发生第二帧头不匹配。
      | 
      | Position=0：还没确认帧头，正在找AA。
      | Position=1：已经见到AA，期望下一个是55。
      | Position≥2：头部已确认，后续字节属于帧内数据。
      | 
      | AA是十六进制，十进制为170；55是十六进制，十进制为85。判断式：
      | 等待AA=(Position==0)；
      | 字节是AA=(Byte==170)；
      | 第二帧头错=(Position==1) AND (Byte!=85)。
      | 
      | 例：Position=1、Byte=AA时，字节是AA和第二帧头错都为真。这并不冲突：它表示没等到55，但可以把这个AA视作重新找头的机会。是否写入、位置如何调整由后面两步分别处理。
      | 
      | 本步骤不检查Active；本字节无效时，后面的写入和位置保持分支会阻止它改变状态。
  Step02_判断本字节能否写入 : Subsystem  Description=|
      | 第二步：决定本字节是否允许写进帧缓存
      | 
      | 收帧必须先找到头，所以不是每个字节都写。将第一步的三个判断与Active组合：
      | 
      | 允许写入=Active AND [
      |   (正在等AA AND 字节是AA)
      |   OR (不在等AA AND 第二帧头没有错)
      | ]。
      | 
      | 分别理解：
      | 还在找AA时，只写AA，其他噪声不进入缓存；
      | 已经见到AA、等待55时，只写正确的55；
      | 头部已经确认后，按顺序接收普通数据，不因数据恰好是AA/55就重新找头；
      | Active为假时，上述条件再合适也不写。
      | 
      | 例：已见AA后又来AA，本步骤不把第二个AA写进第2项；后面的重同步位置逻辑仍保留“已见AA”的状态，继续等55。
      | 
      | 输出只是一项布尔写许可，送第四步。它不产生新缓存，也不判断整帧校验。
  Step03_计算写入位置与是否满帧 : Subsystem  Description=|
      | 第三步：算本次写到第几项，并判断是否到帧尾
      | 
      | Position表示本次之前已接收多少项。本次候选写入位置=Position+1；帧长度固定为22，达到帧尾=(候选写入位置==22)。
      | 
      | 例如Position=0时，候选位置是1，AA应写到第1项；Position=1时，55应写到第2项；Position=21时，本次候选位置是22，这是最后一项。
      | 
      | 注意这里算的是“候选位置”：即使Active为假，仍可计算Position+1，但第四、第五步会保持缓存和位置。不能仅因候选位置等于22就认定收到新帧。
      | 
      | 候选位置送第四步写缓存；它及“达到帧尾”标志也送第五步，决定继续推进还是收齐后回0。本处不保存Position，也不清空缓存。
  Step04_写入字节或保持原缓存 : Subsystem  Description=|
      | 第四步：只更新应写的一项，其他内容保留
      | 
      | 输入包括旧缓存、本次Byte、候选写入位置和写许可。先将索引取min(候选位置,22)，防止索引超过22项缓存上界，再用Assignment生成“把这一项换成Byte”的候选数组。
      | 
      | 最终选择：写许可为真输出更新数组；写许可为假直接输出旧缓存。即使内部算出了候选更新，只要没有许可，它也不会成为输出。
      | 
      | 例：旧位置为5，本次允许接收，就把第6项换成本字节，其他21项保持；若本字节无效或第二帧头错，整份缓存保持。缓存里旧的尾部数据并不会每次清零，所以必须配合Complete和后续校验使用，不能只看数组里有值就当作新帧。
      | 
      | 本步骤不保存跨调用记忆。输出回外层的缓存记忆，供下一个字节/下一批数据继续使用。位置更新与收齐事件在第五步处理。
  Step05_更新收帧位置并报告收齐 : Subsystem  Description=|
      | 第五步：确定下一次收帧位置，并报告刚收齐
      | 
      | 先按收帧阶段选择下一Position：
      | 正在找AA：本字节是AA则到1，否则到0；
      | 正在等55但本字节不匹配：若又是AA则保持1，其他值回0；
      | 正常收数据：未到帧尾就采用Position+1，达到22项后回0，准备找下一帧头。
      | 最后再检查Active：为假时直接保留旧Position，上面的候选变化都不采用。
      | 
      | 收齐事件=Active AND 不在等待第一个AA AND 第二帧头没错 AND 达到22项。
      | 因此它只在有效字节刚补上最后一项时为真，不是缓存里有22项就一直为真。位置回0时，完整缓存仍保留供外层校验。
      | 
      | 例：Position=21，有效字节到来，输出Position=0且Complete=true；同样的位置但Active=false，则输出仍为21且Complete=false。AA、AA、55的序列依次得到位置1、1、2。
      | 
      | 本页不验证CRC或累加/异或校验，也不等待下一个20 ms节拍；Complete交外层决定是否接受这条候选帧。
  Buffer（更新后的帧缓存）_290 : Outport
  Position（下次接收位置）_291 : Outport  Port=2
  Complete（本字节组成完整帧）_292 : Outport  Port=3
  wires:
  Byte（当前字节）_256/1 -> Step04_写入字节或保持原缓存/4(输入4_本项字节), Step01_判断收帧阶段与AA55/1(输入1_本项字节)  "本项字节"
  Step03_计算写入位置与是否满帧/1(输出1_候选位置达到帧长) -> Step05_更新收帧位置并报告收齐/3(输入3_候选位置达到帧长)  "候选位置达到帧长"
  Active（当前字节有效）_257/1 -> Step02_判断本字节能否写入/4(输入4_本项字节有效), Step05_更新收帧位置并报告收齐/2(输入2_本项字节有效)  "本项字节有效"
  Position（已收字节数）_255/1 -> Step03_计算写入位置与是否满帧/1(输入1_本次之前已收字节数), Step01_判断收帧阶段与AA55/2(输入2_本次之前已收字节数), Step05_更新收帧位置并报告收齐/5(输入5_本次之前已收字节数)  "本次之前已收字节数"
  Step01_判断收帧阶段与AA55/1(输出1_当前字节等于AA) -> Step02_判断本字节能否写入/2(输入2_当前字节等于AA), Step05_更新收帧位置并报告收齐/1(输入1_当前字节等于AA)  "当前字节等于AA"
  Step01_判断收帧阶段与AA55/2(输出2_正在寻找第一个AA) -> Step02_判断本字节能否写入/1(输入1_正在寻找第一个AA), Step05_更新收帧位置并报告收齐/6(输入6_正在寻找第一个AA)  "正在寻找第一个AA"
  Step01_判断收帧阶段与AA55/3(输出3_第二帧头不匹配) -> Step02_判断本字节能否写入/3(输入3_第二帧头不匹配), Step05_更新收帧位置并报告收齐/7(输入7_第二帧头不匹配)  "第二帧头不匹配"
  Step03_计算写入位置与是否满帧/2(输出2_候选写入位置) -> Step04_写入字节或保持原缓存/3(输入3_候选写入位置), Step05_更新收帧位置并报告收齐/4(输入4_候选写入位置)  "候选写入位置"
  Step02_判断本字节能否写入/1(输出1_本字节允许写缓存) -> Step04_写入字节或保持原缓存/1(输入1_本字节允许写缓存)  "本字节允许写缓存"
  Buffer（上次收帧缓存）_254/1 -> Step04_写入字节或保持原缓存/2(输入2_上一份候选缓存)  "上一份候选缓存"
  Step05_更新收帧位置并报告收齐/1(输出1_下一次已收字节数) -> Position（下次接收位置）_291/1
  Step05_更新收帧位置并报告收齐/2(输出2_本字节刚收齐) -> Complete（本字节组成完整帧）_292/1
  Step04_写入字节或保持原缓存/1(输出1_更新后的候选缓存) -> Buffer（更新后的帧缓存）_290/1

== system turbo_controller/BoardInput_输入换算与协议解析/In03_Pump（油泵回包预留校验）/Receive（逐字节组帧与保持有效结果）_353/Step03_收齐且校验通过才接受/Verify（完整帧校验）_344 ==
  note: 输入侧预留22字节油泵帧怎样核对CRC
      |
      | Collect送来的是候选完整帧，本模块只在Complete有效时执行校验。内部取协议指定的待校验字节段
      | ，送CRC16逐字节计算，并取出帧尾携带的两个CRC字节。
      |
      | 16位计算结果分为高低两部分：高字节=floor(CRC/256)，低字节=bitand(CRC,255)。分别与帧中对应
      | 位置比较，两项都一致才给出有效结果。
      |
      | 比如计算CRC为十六进制1234，协议中的CRC高字节必须是12、低字节必须是34；顺序反过来也不能通过
      | 。CRC覆盖范围由本页Selector的固定索引决定，不应把帧头或尾部CRC自身随意加入。
      |
      | 输出交给Receive，与“这一轮确实刚收齐一帧”共同决定是否更新反馈。不完整或校验错误时，外层
      | 保留最近有效结果。
      |
      | 本实例CRC覆盖第6～20字节，与第21、22字节的CRC比较。
  Complete（完整帧执行一次）_294 : Inport  OutDataTypeStr=uint32
  Frame（完整候选帧）_296 : Inport  Port=2  OutDataTypeStr=uint8
  CRC16（循环冗余校验）_328 : Subsystem  Description=|
      | 整段字节如何逐个累积CRC16
      | 
      | 这里的输入Bytes是接收帧中由父级Selector选出的数据段。CRC的作用是把整段字节压缩成一个16位检查值，便于接收方发现传输内容变化。
      | 
      | 每帧从初始CRC=uint16(0)开始。循环一次取一个字节，把该字节乘256移到高8位，与旧CRC异或，得到Merged，再交给TableStep执行查表移位。TableStep的输出成为处理下一个字节的旧CRC。
      | 
      | 公式第一步是Merged=bitxor(旧CRC,当前字节×256)。整个循环结束后输出最后一次CRC，父级拆成高、低字节用于比较或发送。For Iterator中的CRC记忆是帧内累积状态，不能理解成跨帧无限累加。
      | 
      | 这里用的是CRC16_Table_Reference指定的算法表，不能随意换另一种CRC表或初始值。相同字节、顺序、表和初值必须得到相同结果，双方才能校验通过。
  Cast（数据类型转换）_329 : DataTypeConversion  OutDataTypeStr=double  RndMeth=Round
  Constant（常量）_330 : Constant  Value=256  OutDataTypeStr=double
  Constant（常量）_334 : Constant  Value=255  OutDataTypeStr=uint16
  Divide（相除）_331 : Product  Inputs=*/  SaturateOnIntegerOverflow=on  OutDataTypeStr=Inherit: Same as first input
  FirstCheck（第一个校验字节一致）_338 : RelationalOperator  Operator===  OutDataTypeStr=boolean  RndMeth=Simplest  InputSameDT=off
  HighByte（高八位）_333 : DataTypeConversion  OutDataTypeStr=uint8  RndMeth=Floor
  LowByte（低八位）_336 : DataTypeConversion  OutDataTypeStr=uint8  RndMeth=Floor
  LowMask（取低八位）_335 : simulink/Logic and Bit Operations/Bitwise Operator  logicop=AND  UseBitMask=off  NumInputPorts=2  BitMask=bin2dec('11011001')  BitMaskRealWorld=Stored Integer
      settings: LibrarySourceBlock=|
      | hdlsllib/Logic and Bit
      | Operations/Bitwise
      | Operator
  Payload（参与循环冗余校验的字节）_297 : Selector  InputPortWidth=22  IndexOptions=Index vector (dialog)  Indices=6:20  OutputSizes=1
  Round（取整）_332 : Rounding
  SecondCheck（第二个校验字节一致）_340 : RelationalOperator  Operator===  OutDataTypeStr=boolean  RndMeth=Simplest  InputSameDT=off
  Select（取指定元素）_337 : Selector  InputPortWidth=22  IndexOptions=Index vector (dialog)  Indices=21  OutputSizes=1
  Select（取指定元素）_339 : Selector  InputPortWidth=22  IndexOptions=Index vector (dialog)  Indices=22  OutputSizes=1
  Valid（两个校验字节均正确）_341 : Logic  IconShape=distinctive  AllPortsSameDT=off  OutDataTypeStr=boolean
  WhenComplete（完整帧才执行一次）_295 : ForIterator  IterationSource=external  ShowIterationPort=off
  Valid（校验是否通过）_342 : Outport
  wires:
  Complete（完整帧执行一次）_294/1 -> WhenComplete（完整帧才执行一次）_295/1  "Complete（完整帧执行一次）"
  Frame（完整候选帧）_296/1 -> Select（取指定元素）_339/1, Select（取指定元素）_337/1, Payload（参与循环冗余校验的字节）_297/1  "Frame（完整候选帧）"
  Payload（参与循环冗余校验的字节）_297/1 -> CRC16（循环冗余校验）_328/1(Bytes（待校验字节）_298)  "Payload（参与循环冗余校验的字节）"
  CRC16（循环冗余校验）_328/1(CRC16（本帧校验结果）_327) -> LowMask（取低八位）_335/1, Cast（数据类型转换）_329/1  "CRC16（循环冗余校验）"
  Cast（数据类型转换）_329/1 -> Divide（相除）_331/1  "Cast（数据类型转换）"
  Constant（常量）_330/1 -> Divide（相除）_331/2  "Constant（常量）"
  Divide（相除）_331/1 -> Round（取整）_332/1  "Divide（相除）"
  Round（取整）_332/1 -> HighByte（高八位）_333/1  "Round（取整）"
  Constant（常量）_334/1 -> LowMask（取低八位）_335/2  "Constant（常量）"
  LowMask（取低八位）_335/1 -> LowByte（低八位）_336/1  "LowMask（取低八位）"
  HighByte（高八位）_333/1 -> FirstCheck（第一个校验字节一致）_338/1  "HighByte（高八位）"
  Select（取指定元素）_337/1 -> FirstCheck（第一个校验字节一致）_338/2  "Select（取指定元素）"
  LowByte（低八位）_336/1 -> SecondCheck（第二个校验字节一致）_340/1  "LowByte（低八位）"
  Select（取指定元素）_339/1 -> SecondCheck（第二个校验字节一致）_340/2  "Select（取指定元素）"
  FirstCheck（第一个校验字节一致）_338/1 -> Valid（两个校验字节均正确）_341/1  "FirstCheck（第一个校验字节一致）"
  SecondCheck（第二个校验字节一致）_340/1 -> Valid（两个校验字节均正确）_341/2  "SecondCheck（第二个校验字节一致）"
  Valid（两个校验字节均正确）_341/1 -> Valid（校验是否通过）_342/1  "Valid（两个校验字节均正确）"

== system turbo_controller/BoardOutput_串口封装与阀门时序/Out01_Pump（泵反馈解析与滤波）/Receive（逐字节组帧与保持有效结果）_680/Step02_拼帧并保存半帧/Collect（帧头识别与缓存推进）_611 ==
  note: 逐字节组帧：本页只做“找帧头、存字节、推进位置”
      |
      | 固定帧长为22字节，帧头是十六进制AA、55。输入为上一份候选缓存、已收字节数Position、本次Byte
      | 和本字节有效Active。输出为更新缓存、下一次使用的Position和本次收齐事件Complete。
      |
      | Position不是本批接收数组的序号：0表示还在找AA，1表示已见AA、正在等55，2～21表示头部已确认
      | 、继续收后面的内容。跨调用的记忆由外层Step02保存，本页根据输入计算一次更新。
      |
      | 按五步看：
      | 1 判断当前是否在等AA或55，以及字节是否匹配。
      | 2 决定这个字节应不应该进入候选缓存。
      | 3 算出本次写入位置Position+1，判断是否达到22。
      | 4 允许写入才更新对应一项，否则保留原缓存。
      | 5 按找头、重同步、收齐和无效字节规则，决定下一位置及Complete。
      |
      | 例：AA→AA→55时，第二个AA保留继续等55的机会，不当作第二帧头写入；头确认后，后续数据即使也
      | 是AA或55，仍按普通数据收下。无效字节不推进位置，也不发收齐事件。
      |
      | Complete仅表示候选帧刚拼满，不表示校验通过；外面的校验步骤还会检查内容。这里没有重写协议或
      | 增加等待时间，五步在同一次字节处理内完成。
  Buffer（上次收帧缓存）_572 : Inport  OutDataTypeStr=uint8
  Position（已收字节数）_573 : Inport  Port=2  OutDataTypeStr=uint16
  Byte（当前字节）_574 : Inport  Port=3  OutDataTypeStr=uint8
  Active（当前字节有效）_575 : Inport  Port=4  OutDataTypeStr=boolean
  Step01_判断收帧阶段与AA55 : Subsystem  Description=|
      | 第一步：看现在收到哪里，并识别AA、55
      | 
      | 只看Position和Byte，不修改缓存，不保存历史。输出三个判断：是否正在找第一个AA、当前字节是否AA、是否发生第二帧头不匹配。
      | 
      | Position=0：还没确认帧头，正在找AA。
      | Position=1：已经见到AA，期望下一个是55。
      | Position≥2：头部已确认，后续字节属于帧内数据。
      | 
      | AA是十六进制，十进制为170；55是十六进制，十进制为85。判断式：
      | 等待AA=(Position==0)；
      | 字节是AA=(Byte==170)；
      | 第二帧头错=(Position==1) AND (Byte!=85)。
      | 
      | 例：Position=1、Byte=AA时，字节是AA和第二帧头错都为真。这并不冲突：它表示没等到55，但可以把这个AA视作重新找头的机会。是否写入、位置如何调整由后面两步分别处理。
      | 
      | 本步骤不检查Active；本字节无效时，后面的写入和位置保持分支会阻止它改变状态。
  Step02_判断本字节能否写入 : Subsystem  Description=|
      | 第二步：决定本字节是否允许写进帧缓存
      | 
      | 收帧必须先找到头，所以不是每个字节都写。将第一步的三个判断与Active组合：
      | 
      | 允许写入=Active AND [
      |   (正在等AA AND 字节是AA)
      |   OR (不在等AA AND 第二帧头没有错)
      | ]。
      | 
      | 分别理解：
      | 还在找AA时，只写AA，其他噪声不进入缓存；
      | 已经见到AA、等待55时，只写正确的55；
      | 头部已经确认后，按顺序接收普通数据，不因数据恰好是AA/55就重新找头；
      | Active为假时，上述条件再合适也不写。
      | 
      | 例：已见AA后又来AA，本步骤不把第二个AA写进第2项；后面的重同步位置逻辑仍保留“已见AA”的状态，继续等55。
      | 
      | 输出只是一项布尔写许可，送第四步。它不产生新缓存，也不判断整帧校验。
  Step03_计算写入位置与是否满帧 : Subsystem  Description=|
      | 第三步：算本次写到第几项，并判断是否到帧尾
      | 
      | Position表示本次之前已接收多少项。本次候选写入位置=Position+1；帧长度固定为22，达到帧尾=(候选写入位置==22)。
      | 
      | 例如Position=0时，候选位置是1，AA应写到第1项；Position=1时，55应写到第2项；Position=21时，本次候选位置是22，这是最后一项。
      | 
      | 注意这里算的是“候选位置”：即使Active为假，仍可计算Position+1，但第四、第五步会保持缓存和位置。不能仅因候选位置等于22就认定收到新帧。
      | 
      | 候选位置送第四步写缓存；它及“达到帧尾”标志也送第五步，决定继续推进还是收齐后回0。本处不保存Position，也不清空缓存。
  Step04_写入字节或保持原缓存 : Subsystem  Description=|
      | 第四步：只更新应写的一项，其他内容保留
      | 
      | 输入包括旧缓存、本次Byte、候选写入位置和写许可。先将索引取min(候选位置,22)，防止索引超过22项缓存上界，再用Assignment生成“把这一项换成Byte”的候选数组。
      | 
      | 最终选择：写许可为真输出更新数组；写许可为假直接输出旧缓存。即使内部算出了候选更新，只要没有许可，它也不会成为输出。
      | 
      | 例：旧位置为5，本次允许接收，就把第6项换成本字节，其他21项保持；若本字节无效或第二帧头错，整份缓存保持。缓存里旧的尾部数据并不会每次清零，所以必须配合Complete和后续校验使用，不能只看数组里有值就当作新帧。
      | 
      | 本步骤不保存跨调用记忆。输出回外层的缓存记忆，供下一个字节/下一批数据继续使用。位置更新与收齐事件在第五步处理。
  Step05_更新收帧位置并报告收齐 : Subsystem  Description=|
      | 第五步：确定下一次收帧位置，并报告刚收齐
      | 
      | 先按收帧阶段选择下一Position：
      | 正在找AA：本字节是AA则到1，否则到0；
      | 正在等55但本字节不匹配：若又是AA则保持1，其他值回0；
      | 正常收数据：未到帧尾就采用Position+1，达到22项后回0，准备找下一帧头。
      | 最后再检查Active：为假时直接保留旧Position，上面的候选变化都不采用。
      | 
      | 收齐事件=Active AND 不在等待第一个AA AND 第二帧头没错 AND 达到22项。
      | 因此它只在有效字节刚补上最后一项时为真，不是缓存里有22项就一直为真。位置回0时，完整缓存仍保留供外层校验。
      | 
      | 例：Position=21，有效字节到来，输出Position=0且Complete=true；同样的位置但Active=false，则输出仍为21且Complete=false。AA、AA、55的序列依次得到位置1、1、2。
      | 
      | 本页不验证CRC或累加/异或校验，也不等待下一个20 ms节拍；Complete交外层决定是否接受这条候选帧。
  Buffer（更新后的帧缓存）_608 : Outport
  Position（下次接收位置）_609 : Outport  Port=2
  Complete（本字节组成完整帧）_610 : Outport  Port=3
  wires:
  Step05_更新收帧位置并报告收齐/2(输出2_本字节刚收齐) -> Complete（本字节组成完整帧）_610/1
  Step05_更新收帧位置并报告收齐/1(输出1_下一次已收字节数) -> Position（下次接收位置）_609/1
  Step04_写入字节或保持原缓存/1(输出1_更新后的候选缓存) -> Buffer（更新后的帧缓存）_608/1
  Step03_计算写入位置与是否满帧/1(输出1_候选位置达到帧长) -> Step05_更新收帧位置并报告收齐/3(输入3_候选位置达到帧长)  "候选位置达到帧长"
  Step03_计算写入位置与是否满帧/2(输出2_候选写入位置) -> Step04_写入字节或保持原缓存/3(输入3_候选写入位置), Step05_更新收帧位置并报告收齐/4(输入4_候选写入位置)  "候选写入位置"
  Buffer（上次收帧缓存）_572/1 -> Step04_写入字节或保持原缓存/2(输入2_上一份候选缓存)  "上一份候选缓存"
  Step02_判断本字节能否写入/1(输出1_本字节允许写缓存) -> Step04_写入字节或保持原缓存/1(输入1_本字节允许写缓存)  "本字节允许写缓存"
  Active（当前字节有效）_575/1 -> Step05_更新收帧位置并报告收齐/2(输入2_本项字节有效), Step02_判断本字节能否写入/4(输入4_本项字节有效)  "本项字节有效"
  Step01_判断收帧阶段与AA55/3(输出3_第二帧头不匹配) -> Step02_判断本字节能否写入/3(输入3_第二帧头不匹配), Step05_更新收帧位置并报告收齐/7(输入7_第二帧头不匹配)  "第二帧头不匹配"
  Step01_判断收帧阶段与AA55/1(输出1_当前字节等于AA) -> Step02_判断本字节能否写入/2(输入2_当前字节等于AA), Step05_更新收帧位置并报告收齐/1(输入1_当前字节等于AA)  "当前字节等于AA"
  Step01_判断收帧阶段与AA55/2(输出2_正在寻找第一个AA) -> Step02_判断本字节能否写入/1(输入1_正在寻找第一个AA), Step05_更新收帧位置并报告收齐/6(输入6_正在寻找第一个AA)  "正在寻找第一个AA"
  Position（已收字节数）_573/1 -> Step03_计算写入位置与是否满帧/1(输入1_本次之前已收字节数), Step05_更新收帧位置并报告收齐/5(输入5_本次之前已收字节数), Step01_判断收帧阶段与AA55/2(输入2_本次之前已收字节数)  "本次之前已收字节数"
  Byte（当前字节）_574/1 -> Step01_判断收帧阶段与AA55/1(输入1_本项字节), Step04_写入字节或保持原缓存/4(输入4_本项字节)  "本项字节"

== system turbo_controller/BoardOutput_串口封装与阀门时序/Out01_Pump（泵反馈解析与滤波）/Receive（逐字节组帧与保持有效结果）_680/Step03_收齐且校验通过才接受/Verify（完整帧校验）_662 ==
  note: 实际22字节油泵反馈怎样核对CRC
      |
      | Collect送来的是候选完整帧，本模块只在Complete有效时执行校验。内部取协议指定的待校验字节段
      | ，送CRC16逐字节计算，并取出帧尾携带的两个CRC字节。
      |
      | 16位计算结果分为高低两部分：高字节=floor(CRC/256)，低字节=bitand(CRC,255)。分别与帧中对应
      | 位置比较，两项都一致才给出有效结果。
      |
      | 比如计算CRC为十六进制1234，协议中的CRC高字节必须是12、低字节必须是34；顺序反过来也不能通过
      | 。CRC覆盖范围由本页Selector的固定索引决定，不应把帧头或尾部CRC自身随意加入。
      |
      | 输出交给Receive，与“这一轮确实刚收齐一帧”共同决定是否更新反馈。不完整或校验错误时，外层
      | 保留最近有效结果。
      |
      | 本实例CRC覆盖第6～20字节，与第21、22字节的CRC比较。
  Complete（完整帧执行一次）_612 : Inport  OutDataTypeStr=uint32
  Frame（完整候选帧）_614 : Inport  Port=2  OutDataTypeStr=uint8
  CRC16（循环冗余校验）_646 : Subsystem  Description=|
      | 整段字节如何逐个累积CRC16
      | 
      | 这里的输入Bytes是接收帧中由父级Selector选出的数据段。CRC的作用是把整段字节压缩成一个16位检查值，便于接收方发现传输内容变化。
      | 
      | 每帧从初始CRC=uint16(0)开始。循环一次取一个字节，把该字节乘256移到高8位，与旧CRC异或，得到Merged，再交给TableStep执行查表移位。TableStep的输出成为处理下一个字节的旧CRC。
      | 
      | 公式第一步是Merged=bitxor(旧CRC,当前字节×256)。整个循环结束后输出最后一次CRC，父级拆成高、低字节用于比较或发送。For Iterator中的CRC记忆是帧内累积状态，不能理解成跨帧无限累加。
      | 
      | 这里用的是CRC16_Table_Reference指定的算法表，不能随意换另一种CRC表或初始值。相同字节、顺序、表和初值必须得到相同结果，双方才能校验通过。
  Cast（数据类型转换）_647 : DataTypeConversion  OutDataTypeStr=double  RndMeth=Round
  Constant（常量）_648 : Constant  Value=256  OutDataTypeStr=double
  Constant（常量）_652 : Constant  Value=255  OutDataTypeStr=uint16
  Divide（相除）_649 : Product  Inputs=*/  SaturateOnIntegerOverflow=on  OutDataTypeStr=Inherit: Same as first input
  FirstCheck（第一个校验字节一致）_656 : RelationalOperator  Operator===  OutDataTypeStr=boolean  RndMeth=Simplest  InputSameDT=off
  HighByte（高八位）_651 : DataTypeConversion  OutDataTypeStr=uint8  RndMeth=Floor
  LowByte（低八位）_654 : DataTypeConversion  OutDataTypeStr=uint8  RndMeth=Floor
  LowMask（取低八位）_653 : simulink/Logic and Bit Operations/Bitwise Operator  logicop=AND  UseBitMask=off  NumInputPorts=2  BitMask=bin2dec('11011001')  BitMaskRealWorld=Stored Integer
      settings: LibrarySourceBlock=|
      | hdlsllib/Logic and Bit
      | Operations/Bitwise
      | Operator
  Payload（参与循环冗余校验的字节）_615 : Selector  InputPortWidth=22  IndexOptions=Index vector (dialog)  Indices=6:20  OutputSizes=1
  Round（取整）_650 : Rounding
  SecondCheck（第二个校验字节一致）_658 : RelationalOperator  Operator===  OutDataTypeStr=boolean  RndMeth=Simplest  InputSameDT=off
  Select（取指定元素）_655 : Selector  InputPortWidth=22  IndexOptions=Index vector (dialog)  Indices=21  OutputSizes=1
  Select（取指定元素）_657 : Selector  InputPortWidth=22  IndexOptions=Index vector (dialog)  Indices=22  OutputSizes=1
  Valid（两个校验字节均正确）_659 : Logic  IconShape=distinctive  AllPortsSameDT=off  OutDataTypeStr=boolean
  WhenComplete（完整帧才执行一次）_613 : ForIterator  IterationSource=external  ShowIterationPort=off
  Valid（校验是否通过）_660 : Outport
  wires:
  Complete（完整帧执行一次）_612/1 -> WhenComplete（完整帧才执行一次）_613/1  "Complete（完整帧执行一次）"
  Frame（完整候选帧）_614/1 -> Select（取指定元素）_657/1, Select（取指定元素）_655/1, Payload（参与循环冗余校验的字节）_615/1  "Frame（完整候选帧）"
  Payload（参与循环冗余校验的字节）_615/1 -> CRC16（循环冗余校验）_646/1(Bytes（待校验字节）_616)  "Payload（参与循环冗余校验的字节）"
  CRC16（循环冗余校验）_646/1(CRC16（本帧校验结果）_645) -> LowMask（取低八位）_653/1, Cast（数据类型转换）_647/1  "CRC16（循环冗余校验）"
  Cast（数据类型转换）_647/1 -> Divide（相除）_649/1  "Cast（数据类型转换）"
  Constant（常量）_648/1 -> Divide（相除）_649/2  "Constant（常量）"
  Divide（相除）_649/1 -> Round（取整）_650/1  "Divide（相除）"
  Round（取整）_650/1 -> HighByte（高八位）_651/1  "Round（取整）"
  Constant（常量）_652/1 -> LowMask（取低八位）_653/2  "Constant（常量）"
  LowMask（取低八位）_653/1 -> LowByte（低八位）_654/1  "LowMask（取低八位）"
  HighByte（高八位）_651/1 -> FirstCheck（第一个校验字节一致）_656/1  "HighByte（高八位）"
  Select（取指定元素）_655/1 -> FirstCheck（第一个校验字节一致）_656/2  "Select（取指定元素）"
  LowByte（低八位）_654/1 -> SecondCheck（第二个校验字节一致）_658/1  "LowByte（低八位）"
  Select（取指定元素）_657/1 -> SecondCheck（第二个校验字节一致）_658/2  "Select（取指定元素）"
  FirstCheck（第一个校验字节一致）_656/1 -> Valid（两个校验字节均正确）_659/1  "FirstCheck（第一个校验字节一致）"
  SecondCheck（第二个校验字节一致）_658/1 -> Valid（两个校验字节均正确）_659/2  "SecondCheck（第二个校验字节一致）"
  Valid（两个校验字节均正确）_659/1 -> Valid（校验是否通过）_660/1  "Valid（两个校验字节均正确）"

== system turbo_controller/BoardOutput_串口封装与阀门时序/Out04_Command（电机及油泵指令）/MotorFrame（电机指令高字节固定为零）_925/CRC16（只校验两个命令字节）_912/TableStep（查表更新本字节校验） ==
  note: 【中文学习说明：一次查表更新一个字节】
      | 一、输入已经是“旧CRC XOR (当前字节×256)”。
      | 输入是16位无符号整数，记作Merged（合并值）。
      |
      | 二、上路得到查表下标。
      | 合并值÷256后向下取整，取得高八位，范围0～255。
      | 这等价于参考程序中的“旧CRC高字节 XOR 当前字节”。
      | Lookup（按下标取表项）采用Zero-based（从0编号），
      | 所以0就取表的第一项，255取最后一项，不能再加1。
      |
      | 三、下路准备左移结果。
      | 先转uint32（32位无符号数），再乘256左移8位，
      | 与65535作按位AND，只保留低16位，最后转回uint16。
      | 先加宽再移位，是为了避免整数饱和破坏结果。
      | 当前字节已经在高8位，左移后移出16位范围，
      | 因此截断后与“旧CRC左移8位”的结果相同。
      |
      | 四、两路按位XOR（异或），输出更新后的16位CRC。
      | 异或的意思：两个二进制位相同得0，不同得1。
      | 本页不需要循环和记忆，输入一到就能按组合逻辑计算；
      | 跨字节的累计和每帧初值由父级CRC16模块负责。
      |
      | 五、CRC16Table（查表数据）是256项整数常量。
      | 表内容逐项复制自参考工程USER/crc.c，
      | 与NRIST_lib/NRIST_calculate.c中的表一致。
      | Selector（按下标选取）直接取一项，不做曲线插值。
      | 表中数值不是需要现场调节的控制参数。
  note: CRC16的一个字节怎样查表更新
      |
      | 父级已经把当前数据字节异或进旧CRC的高8位，形成Merged。本模块把这个16位数拆成“用哪项表”和
      | “保留哪些移位结果”两部分。
      |
      | 先取高8位：索引=floor(Merged/256)，范围0～255。用它到CRC16_Table_Reference查表；模型Select
      | or按零基索引取值，写成MATLAB数组下标时要用索引+1。
      | 另一条支路把Merged左移一个字节，即乘256，然后只保留低16位：移位值=bitand(uint32(Merged)×25
      | 6,65535)。
      |
      | 最后将表值与移位值按位异或：
      | 新CRC=bitxor(表值,移位值)。
      |
      | 例如Merged=十六进制1234，高8位12用于选表项，左移并截16位后为3400，再与表项异或。宽类型uint
      | 32是为了中间计算不先溢出，并不表示输出CRC变成32位。结果回到父级，继续处理下一个数据字节。
  Merged（旧校验值与当前字节异或后的数） : Inport  OutDataTypeStr=uint16
  CRC16Table（参考工程原始二百五十六项表） : Constant  Value=CRC16_Table_Reference  OutDataTypeStr=uint16
  Divisor（高字节换算除数） : Constant  Value=256  OutDataTypeStr=double
  Exact（转双精度做精确除法） : DataTypeConversion  OutDataTypeStr=double  SaturateOnIntegerOverflow=off  RndMeth=Floor
  HighByte（除二百五十六取高字节） : Product  Inputs=*/  OutDataTypeStr=double
  Index（向下取整得到零至二百五十五） : DataTypeConversion  OutDataTypeStr=uint32  RndMeth=Floor
  LeftByte（左移一个字节） : Product  Inputs=**  OutDataTypeStr=uint32  SaturateOnIntegerOverflow=on
  Lookup（按零基索引读取校验表） : Selector  IndexMode=Zero-based  InputPortWidth=256  IndexOptions=Index vector (port)  Indices=1  OutputSizes=1
  Mask16（保留低十六位） : Constant  Value=65535  OutDataTypeStr=uint32
  Shift16（移位结果转十六位） : DataTypeConversion  OutDataTypeStr=uint16  SaturateOnIntegerOverflow=off  RndMeth=Floor
  ShiftBase（一个字节的移位系数） : Constant  Value=256  OutDataTypeStr=uint32
  Update（查表值与移位结果异或） : simulink/Logic and Bit Operations/Bitwise Operator  logicop=XOR  UseBitMask=off  NumInputPorts=2  BitMask=bin2dec('11011001')  BitMaskRealWorld=Stored Integer
      settings: LibrarySourceBlock=|
      | hdlsllib/Logic and Bit
      | Operations/Bitwise
      | Operator
  Wide（转三十二位防止移位溢出） : DataTypeConversion  OutDataTypeStr=uint32  SaturateOnIntegerOverflow=off  RndMeth=Floor
  Wrap16（截取左移后的低十六位） : simulink/Logic and Bit Operations/Bitwise Operator  logicop=AND  UseBitMask=off  NumInputPorts=2  BitMask=bin2dec('11011001')  BitMaskRealWorld=Stored Integer
      settings: LibrarySourceBlock=|
      | hdlsllib/Logic and Bit
      | Operations/Bitwise
      | Operator
  CRC（本字节处理后的校验值） : Outport
  wires:
  Update（查表值与移位结果异或）/1 -> CRC（本字节处理后的校验值）/1
  Shift16（移位结果转十六位）/1 -> Update（查表值与移位结果异或）/2
  Lookup（按零基索引读取校验表）/1 -> Update（查表值与移位结果异或）/1
  Index（向下取整得到零至二百五十五）/1 -> Lookup（按零基索引读取校验表）/2
  CRC16Table（参考工程原始二百五十六项表）/1 -> Lookup（按零基索引读取校验表）/1
  HighByte（除二百五十六取高字节）/1 -> Index（向下取整得到零至二百五十五）/1
  Divisor（高字节换算除数）/1 -> HighByte（除二百五十六取高字节）/2
  Exact（转双精度做精确除法）/1 -> HighByte（除二百五十六取高字节）/1
  Wrap16（截取左移后的低十六位）/1 -> Shift16（移位结果转十六位）/1
  Mask16（保留低十六位）/1 -> Wrap16（截取左移后的低十六位）/2
  LeftByte（左移一个字节）/1 -> Wrap16（截取左移后的低十六位）/1
  ShiftBase（一个字节的移位系数）/1 -> LeftByte（左移一个字节）/2
  Wide（转三十二位防止移位溢出）/1 -> LeftByte（左移一个字节）/1
  Merged（旧校验值与当前字节异或后的数）/1 -> Exact（转双精度做精确除法）/1, Wide（转三十二位防止移位溢出）/1
